simulink model "tc_dynamic_rl"  (R2026b)
settings: Solver=ode15s  StopTime=0.0015  MaxStep=1.9999999999999999e-07  RelTol=1e-06  AbsTol=1e-09
model workspace (MAT data in the model file):
  tcCommand = timeseries
  tcCommand.Name = 'unnamed'
  tcCommand.DataInfo = tsdata.datametadata
  tcCommand.DataInfo.Interpolation = tsdata.interpolation
  tcCommand.DataInfo.Interpolation.Fhandle : function handle (value not decoded)
  tcCommand.DataInfo.Interpolation.Name = 'linear'
  tcCommand.TimeInfo = tsdata.timemetadata
  tcCommand.TimeInfo.Length = 6
  tcCommand.TimeInfo.DuplicateTimes = 0
  tcCommand.TimeInfo.Time_ = [0; 5e-05; 0.0003; 0.0004; 0.0005; 0.0015]
  tcCommand.TimeInfo.Initialized = 1
  tcCommand.QualityInfo = tsdata.qualmetadata
  tcCommand.Data_ = [0; 1; 0; 1; 0; 0]
libraries: fl_lib x15, nesl_utility x10, ee_lib x3
settings Model: Creator=ganib  LastModifiedBy=ganib
settings SimscapeCC: SimscapeLogType=all  SimscapeNominalValues="[{\"value\":\"1\",\"unit\":\"A\"},{\"value\":\"1\",\"unit\":\"bar\"},{\"value\":\"1\",\"unit\":\"cm^2\"},{\"value\":\"1\",\"unit\":\"cm^3/s\"},{\"value\":\"1\",\"unit\":\"kJ/kg\"},{\"value\":\"1\",\"unit\":\"kW\"},{\"value\":\"1\",\"unit\":\"l\"},{\"value\":\"1\",\"unit\":\"N\"},{\"value\":\"1\",\"unit\":\"N*m\"},{\"value\":\"1\",\"unit\":\"V\"},{\"value\":\"0.001\",\"unit\":\"Wb\"}]"  SimscapeUseEnergyAccounting=off

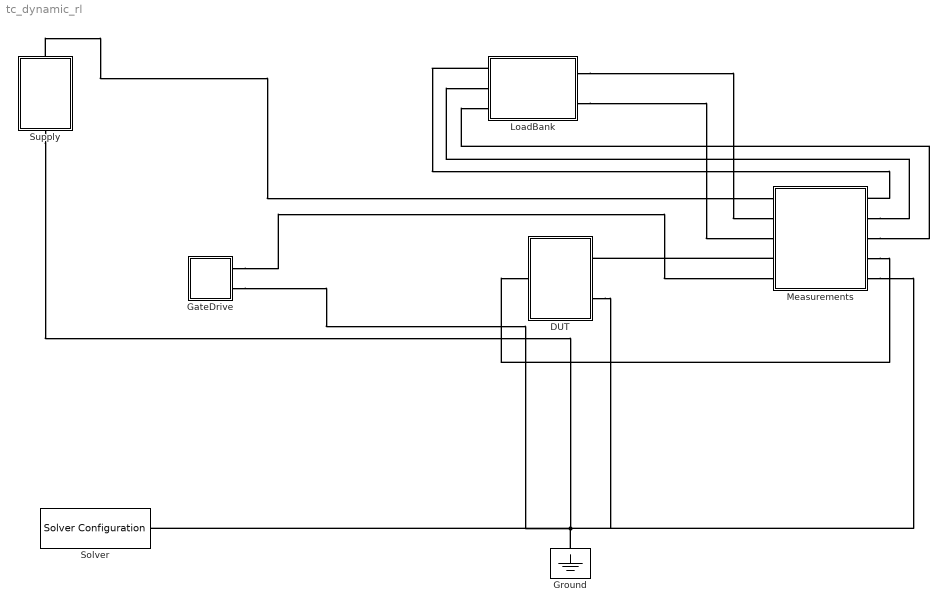
== system tc_dynamic_rl ==
  DUT : Subsystem
  GateDrive : Subsystem
  Ground : fl_lib/Electrical/Electrical Elements/Electrical Reference
  LoadBank : Subsystem
  Measurements : Subsystem
  Solver : nesl_utility/Solver Configuration  PhysicalDomain=network_engine_domain  SubClassName=solver  LeftPortType=input  RightPortType=generic  Tones=[]  Harmonics=[]  SimulateNoise=off  Profile=off  UseLocalSampling=off  EnableSwitchedLinearOptims=on  FrequencyDomain=off  UseCCode=off  RelTol=0.001  AbsTol=0.001  MinStep=1e-09  ToWorkspace=off  RevertToSquareIcSolve=off  NumHomotopyIterations=100  PhasorMode=off  PhasorModeNumHarmonics=1  ConsistencySolver=NEWTON_XTOL_AFTER_FTOL  CanonicalOrdering=CANONICAL  OptimizeIntermediates=OPTIMIZED  MulticoreSolverChoice=BACKWARD_EULER  IndexReductionMethod=DerivativeReplacement  DoDC=on  ResidualTolerance=1e-09  ConsistencyTolSource=GLOBAL  ConsistencyAbsTol=0.001  ConsistencyRelTol=0.001  ConsistencyTolFactor=0.001  UseLocalSolver=off  LocalSolverChoice=NE_BACKWARD_EULER_ADVANCER  ResolveIndetEquations=on  FunctionEvalNumThread=1  LocalSolverSampleTime=0.001  DoFixedCost=off  MaxNonlinIter=3  MaxModeIter=2  ComputeImpulses=off  ImpulseIterations=2  LinearAlgebra=auto  LinearAlgebraNumThread=0  EquationFormulation=NE_TIME_EF  DelaysMemoryBudget=1024  AutomaticFiltering=on  FilteringTimeConstant=0.001  PartitionStorageMethod=AS_NEEDED  PartitionMemoryBudget=1024  PartitionMethod=BALANCED  MultibodyUseLocalSolver=off  MultibodyLocalSolverChoice=ODE1  MultibodyLocalSolverSampleTime=0.001
  Supply : Subsystem
  connections:
  Ground/LConn1 -- Supply/RConn1 -- Measurements/RConn5 -- DUT/RConn2 -- GateDrive/RConn2 -- Solver/RConn1
  Supply/LConn1 -- Measurements/LConn1
  LoadBank/LConn1 -- Measurements/RConn1
  LoadBank/RConn1 -- Measurements/LConn2
  Measurements/RConn2 -- LoadBank/LConn2
  LoadBank/RConn2 -- Measurements/LConn3
  Measurements/RConn3 -- LoadBank/LConn3
  Measurements/LConn4 -- DUT/RConn1
  GateDrive/RConn1 -- Measurements/LConn5
  Measurements/RConn4 -- DUT/LConn1

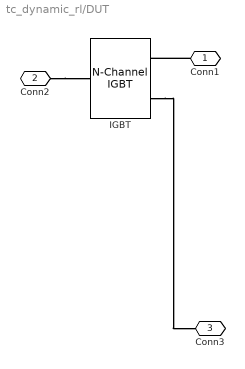
== system tc_dynamic_rl/DUT ==
  IGBT : ee_lib/Semiconductors & Converters/N-Channel IGBT  model_type=ee.enum.igbt.parameterization.equation  Ices=1.1501079949162614e-07 A  Vces=3300 V  Vth=6.3 V  Vce_sat=2.6 V  Ice_sat=1500 A  Vge_sat=15 V  Tmeas=25 degC  Vge_vec=[-1, 0, 2, 3, 5, 6, 7, 8, 10, 12, 15, 18, 20] V  Vce_vec=[0, .25, .5, .75, 1, 1.26, 1.51, 1.76, 2.01, 2.26, 2.51, 2.76, 3.01, 3.27, 3.52, 3.77, 4.02, 4.27, 4.52, 4.77] V  T_vec=[25, 125] degC  Ic_mat=[0, 0, 0, 0, 0, 0, 0, 0, 0, 0, 0, 0, 0, 0, 0, 0, 0, 0, 0, 0; 0, 0, 0, 0, 0, 0, 0, 0, 0, 0, 0, 0, 0, 0, 0, 0, 0, 0, 0, 0; 0, 0, 0, 0, 0, 0, 0, 0, 0, 0, 0, 0, 0, 0, 0, 0, 0, 0, 0, 0; 0, 0, 0, 0, 0, 0, 0, 0, 0, 0, 0, 0, 0, 0, 0, 0, 0, 0, 0, 0; 0, 0, 0, 0, 0, 0, 0, 0, 0, 0, 0, 0, 0, 0, 0, 0, 0, 0, 0, 0; 0, 0, 0, .81, 3.13, 4.97, 6.03, 6.53, 6.84, 7.01, 7.19, 7.32, 7.44, 7.55, 7.67, 7.78, 7.89, 8, 8.07, 8.07; 0, 0, 0, 1.07, 5.5, 12.93, 22.09, 29.14, 35.27, 38.97, 41.37, 43.08, 44.52, 45.45, 46.28, 46.85, 47.41, 47.76, 48.06, 48.36; 0, 0, 0, 1.1, 6.99, 16.51, 28.38, 41.53, 55.76, 69.08, 80.5, 89.56, 96.13, 101.45, 105.15, 107.99, 110.09, 111.87, 113.54, 114.95; 0, 0, 0, 1.36, 6.26, 17.43, 33.6, 50.43, 71.75, 93.61, 114.64, 134.42, 151.44, 164.25, 177.06, 189.88, 202.69, 215.51, 228.32, 241.14; 0, 0, 0, 1.42, 6.4, 18.7, 36.19, 55.23, 79.71, 106.22, 131.28, 156.62, 182.79, 208.97, 235.15, 261.32, 287.5, 313.67, 339.85, 366.02; 0, 0, 0, 1.45, 6.81, 20.01, 39.61, 60.63, 88.74, 117.7, 147.16, 191.87, 237.14, 282.42, 327.69, 372.96, 418.23, 463.5, 508.77, 554.04; 0, 0, 0, 1.49, 6.97, 20.55, 41.34, 64.15, 94.91, 126.1, 170.16, 233.77, 297.38, 360.98, 424.59, 488.19, 551.8, 615.4, 679.01, 742.62; 0, 0, 0, 1.5, 7.5, 20.96, 42.17, 66.19, 98.34, 131.14, 187.84, 263.46, 339.09, 414.72, 490.34, 565.97, 641.6, 717.22, 792.85, 868.48] A  Ic_mat_3D=zeros(13, 20, 2) A  C_param=ee.enum.igbt.capacitanceParam.fixedciss  C_GE=23.7 nF  C_GC=2.7 nF  C_CE=0 nF  C_ies=1.6400000000000001e-07 F  C_res=1.3999999999999999e-09 F  C_oes=1.0999999999999999e-08 F  C_GE_vec=[25, 31, 26.5, 24.9, 25, 24.9, 24.6, 24.7, 24.8] nF  C_GC_vec=[55, 9, 5.5, 3.1, 2.5, 2.1, 1.9, 1.8, 1.7] nF  C_Vge_vec=0 V  C_CE_vec=[5, 11, 6.5, 4.9, 3.5, 2.7, 2.1, 1.7, 1.4] nF  C_ies_vec=[80, 40, 32, 28, 27.5, 27, 26.5, 26.5, 26.5] nF  C_res_vec=[55, 9, 5.5, 3.1, 2.5, 2.1, 1.9, 1.8, 1.7] nF  C_oes_vec=[60, 20, 12, 8, 6, 4.8, 4, 3.5, 3.1] nF  C_Vce_vec=[0, 1, 2, 5, 10, 15, 20, 25, 30] V  charge_linearity_param=ee.enum.igbt.cgcLinearity.constant  C_OX=20 nF  V_C_OX=-5 V  TF=1.9999999999999999e-07 s  TT=0 us  LeadRc=0 Ohm  LeadRe=0 Ohm  LeadRg=0 Ohm  LC=0 nH  LE=0 nH  LG=0 nH  ec=1  VAF=200 V  RC=4.5e-05 Ohm  RE=4.5e-05 Ohm  RG=0.5 Ohm  BF=50  T_param=ee.enum.igbt.temperatureParameterization.IcesVce  Ices_T2=0.0040000000000000001 A  EG=1.11 eV  Vce_sat_T2=3.2 V  Tmeas2=125 degC  XTI=3  BEX=-1.5  RG_alpha=0 1/K  Tdevice=25 degC  Tdevice_3D=25 degC  ig_specify=off  ig_priority=None  ig=0 A  ig_nominal_specify=off  ig_nominal_value=1  ig_nominal_unit=A  ic_specify=off  ic_priority=None  ic=0 A  ic_nominal_specify=off  ic_nominal_value=1  ic_nominal_unit=A  vge_specify=off  vge_priority=None  vge=0 V  vge_nominal_specify=off  vge_nominal_value=1  vge_nominal_unit=V  vce_specify=off  vce_priority=None  vce=0 V  vce_nominal_specify=off  vce_nominal_value=1  vce_nominal_unit=V  v_Cge_specify=off  v_Cge_priority=High  v_Cge=0 V  v_Cge_nominal_specify=off  v_Cge_nominal_value=1  v_Cge_nominal_unit=V  v_Cce_specify=off  v_Cce_priority=High  v_Cce=0 V  v_Cce_nominal_specify=off  v_Cce_nominal_value=1  v_Cce_nominal_unit=V  thermal_network_parameterization=ee.enum.thermalNetworkTopology.junctionCase  Rth=[0, 10] K/W  Rth_Cauer=[1, 3, 10] K/W  Rth_Foster=[.08, .14, .22, .16] K/W  thermal_mass_parameterization=ee.enum.thermalNetwork.timeconstant  thermal_mass=[0, 1] J/K  thermal_mass_Cauer=[.1, .3, 1] J/K  thermal_mass_Foster=[.001, .005, .05, .5] J/K  thermal_time_constant=[0, 10] s  thermal_time_constant_Cauer=[1, 3, 10] s  thermal_time_constant_Foster=[7e-05, .0007, .01, .08] s  thermal_mass_initial_temperatures=[25, 25] degC  thermal_mass_initial_temperatures_Cauer=[25, 25, 25] degC  Tvec_initial_Foster=[25, 25, 25, 25] degC  Ic_vec1=[0, 10, 50, 100, 200, 400, 600] A  Vce_vec1=[0, 1.1, 1.3, 1.45, 1.75, 2.25, 2.7] V  Rmiller=0.1 Ohm  Goff=1e-5 1/Ohm  t_on=0.07 us  t_rise=0.7 us  t_off=0.2 us  t_fall=0.5 us  v_meas=300 V  vStartTurnOn_specify=off  vStartTurnOn_priority=None  vStartTurnOn=1 V  tStartTurnOn_specify=off  tStartTurnOn_priority=None  tStartTurnOn=0 s  vStartTurnOff_specify=off  vStartTurnOff_priority=None  vStartTurnOff=0.5 V  tStartTurnOff_specify=off  tStartTurnOff_priority=None  tStartTurnOff=0 s  Tj_vec1=[298.15, 398.15] K  Vce_mat1=[0, 1.1, 1.3, 1.45, 1.75, 2.25, 2.7; 0, 1, 1.15, 1.35, 1.7, 2.35, 3] V  Tj_vec_loss=[298.15, 398.15] K  Ic_vec_loss=[0, 10, 50, 100, 200, 400, 600] A  E_turn_on_mat1=[0, .2, 1, 2, 4, 8, 15; 0, .3, 1.3, 2.5, 5, 11, 18] * 1e-3 J  E_turn_off_mat1=[0, .3, 1.5, 3, 6, 15, 25; 0, .7, 3.3, 6.5, 13, 25, 35] * 1e-3 J  iStartTurnOff_specify=off  iStartTurnOff_priority=None  iStartTurnOff=0 A  Tdevice_specify=off  Tdevice_priority=None
  Conn1 : PMIOPort  Side=Right
  Conn2 : PMIOPort  Port=2  Side=Left
  Conn3 : PMIOPort  Port=3  Side=Right
  connections:
  Conn1/RConn1 -- IGBT/RConn1
  Conn2/RConn1 -- IGBT/LConn1
  IGBT/RConn2 -- Conn3/RConn1

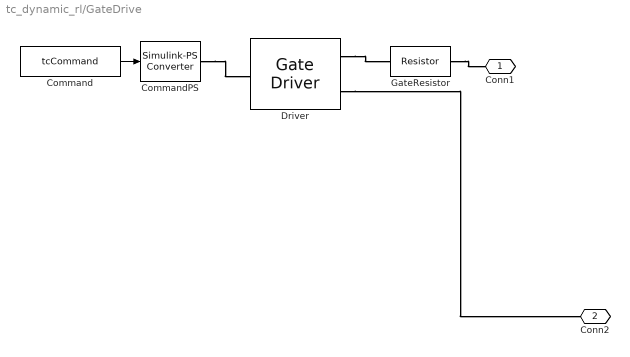
== system tc_dynamic_rl/GateDrive ==
  Command : FromWorkspace  VariableName=tcCommand  Interpolate=off  OutputAfterFinalValue=Holding final value
  CommandPS : nesl_utility/Simulink-PS Converter  PhysicalDomain=network_engine_domain  SubClassName=ps_input  LeftPortType=input  RightPortType=output  PseudoPeriodic=off  Frequencies=[]  NoiseDistribution=none  NoiseParameters=[]  Unit=1  AffineConversion=off  FilteringAndDerivatives=zero  SimscapeFilterOrder=1  InputFilterTimeConstant=0.001  UdotUserProvided=0
  Driver : ee_lib/Semiconductors & Converters/Gate Driver  port_option=ee.enum.controlport.ps  uHigh=2.0 V  uLow=0.8 V  uHighValue=0.7  uLowValue=0.3  vHigh=12 V  vLow=-15 V  tHigh=4.9999999999999998e-08 s  tLow=4.9999999999999998e-08 s  parameterization=ee.enum.semiconductors.gateDriverParam.outputImpedance  rHigh=2 Ohm  rLow=27 Ohm  tRise=20 ns  tFall=20 ns  cLoad=10 nF  ZonTime_specify=off  ZonTime_priority=None  ZonTime=0 s  ZoffTime_specify=off  ZoffTime_priority=None  ZoffTime=0 s
  GateResistor : fl_lib/Electrical/Electrical Elements/Resistor  R=0 Ohm  i_specify=off  i_priority=None  i=0 A  i_nominal_specify=off  i_nominal_value=1  i_nominal_unit=A  v_specify=off  v_priority=None  v=0 V  v_nominal_specify=off  v_nominal_value=1  v_nominal_unit=V
  Conn1 : PMIOPort  Side=Right
  Conn2 : PMIOPort  Port=2  Side=Right
  wires:
  Command/1 -> CommandPS/1
  connections:
  Driver/RConn1 -- GateResistor/LConn1
  CommandPS/RConn1 -- Driver/LConn1
  GateResistor/RConn1 -- Conn1/RConn1
  Driver/RConn2 -- Conn2/RConn1

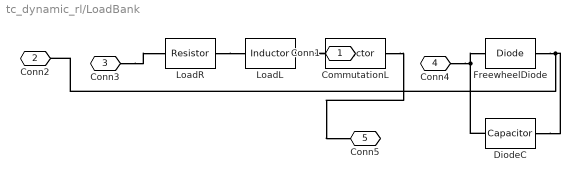
== system tc_dynamic_rl/LoadBank ==
  CommutationL : fl_lib/Electrical/Electrical Elements/Inductor  l=9.9999999999999995e-08 H  r=0.0001 Ohm  g=0 1/Ohm  i_specify=off  i_priority=None  i=0 A  i_nominal_specify=off  i_nominal_value=1  i_nominal_unit=A  v_specify=off  v_priority=None  v=0 V  v_nominal_specify=off  v_nominal_value=1  v_nominal_unit=V  i_L_specify=off  i_L_priority=High  i_L=0 A  i_L_nominal_specify=off  i_L_nominal_value=1  i_L_nominal_unit=A
  DiodeC : fl_lib/Electrical/Electrical Elements/Capacitor  c=1.0999999999999999e-08 F  r=1e-6 Ohm  g=0 1/Ohm  i_specify=off  i_priority=None  i=0 A  i_nominal_specify=off  i_nominal_value=1  i_nominal_unit=A  v_specify=off  v_priority=None  v=0 V  v_nominal_specify=off  v_nominal_value=1  v_nominal_unit=V  vc_specify=off  vc_priority=High  vc=0 V  vc_nominal_specify=off  vc_nominal_value=1  vc_nominal_unit=V
  FreewheelDiode : ee_lib/Semiconductors & Converters/Diode  Vf=0.5 V  Ron=0.0012 Ohm  Goff=1e-08 S  N_series=1  N_parallel=1  ZenerEnable=false  BV=30 V  Rz=0.3 Ohm  enable_fault_composite=simscape.enum.onoff.off  i_specify=off  i_priority=None  i=0 A  i_nominal_specify=off  i_nominal_value=1  i_nominal_unit=A  v_specify=off  v_priority=None  v=0 V  v_nominal_specify=off  v_nominal_value=1  v_nominal_unit=V  ModelType=ee.enum.diode.idealModelType.pwl  TableType=ee.enum.diode.tableType.IfMat  IfMat=[.07, .12, .19, 1.75, 4.24, 7.32, 11.2; .16, .3, .72, 2.14, 5.02, 8.35, 13.12] A  VfMat=[.9, 1.15, 1.25, 1.5, 1.75, 2.17, 2.6, 2.85; .58, .68, .75, 1.1, 1.38, 1.77, 2.27, 2.7] V  TjVec=[25, 125] degC  VfVec=[.5, .7, .9, 1.3, 1.7, 2.1, 2.5] V  IfVec=[.1, .2, .5, 1, 2, 4, 7, 10] A  IrMat=[1e-06, 2e-06, 5e-06, 1e-05, 2.5e-05, 5e-05, .0001; 2e-06, 5e-06, 1e-05, 4e-05, 8e-05, .0002, .0005] A  VrMat=[10, 100, 200, 250, 300, 325, 350; 10, 70, 160, 220, 270, 300, 320] V  VrVec=[10, 20, 40, 50, 70, 80, 100] V  IrVec=[1e-06, 2e-06, 5e-06, 1e-05, 2e-05, 5e-05, .0001] A  rec_loss_model=ee.enum.diode.reverseRecoveryModelTabulateUpTo3D.fixed  ErecVal=0 J  scaleWithIandV=true  ErecMat=zeros(2, 3) J  ErecMat3D=zeros(2, 3, 2) J  TjrecVec=[25, 125] degC  IfrecVec=[.1, 1, 10] A  IrecVal=10 A  VrecVal=10 V  VrecVec=[0, 100] V  tFilter=1 / 1000 / 100 s  thermal_network_parameterization=ee.enum.thermalNetworkTopology.junctionCase  Rth=[0, 10] K/W  Rth_Cauer=[1, 3, 10] K/W  Rth_Foster=[.08, .14, .22, .16] K/W  thermal_mass_parameterization=ee.enum.thermalNetwork.timeconstant  thermal_mass=[0, 1] J/K  thermal_mass_Cauer=[.1, .3, 1] J/K  thermal_mass_Foster=[.001, .005, .05, .5] J/K  thermal_time_constant=[0, 10] s  thermal_time_constant_Cauer=[1, 3, 10] s  thermal_time_constant_Foster=[7e-05, .0007, .01, .08] s  thermal_mass_initial_temperatures=[25, 25] degC  thermal_mass_initial_temperatures_Cauer=[25, 25, 25] degC  thermal_mass_initial_temperatures_Foster=[25, 25, 25, 25] degC  junction_thermal_mass=0.01 J/K  junction_temperature_specify=off  junction_temperature_priority=None  junction_temperature=25 degC  junction_temperature_nominal_specify=off  junction_temperature_nominal_value=1  junction_temperature_nominal_unit=degC  ThermalPort=false  ModelTypePhysical=ee.enum.diode.physicalModelType.exponential  prmExp=ee.enum.diode.expParam.useTwo  I12=[.0137, .545] A  V12=[.6, .7] V  IS=1e-12 A  ec=1  I1=0.0137 A  V1=0.6 V  RS=0 Ohm  C_param=ee.enum.diode.capParam.fixed  CJ=0 pF  CJ0=5 pF  Vvec=[.1, 10, 100] V  Cvec=[3.5, 1, .4] pF  VJ=1 V  Mgrad=0.5  FC=0.5  Q_param=ee.enum.diode.recoveryParam.off  iRM=-7.15 A  iF=4 A  didt=-750 A/us  trr_factor=3  trr=115 ns  Qrr=150 nA*s  Vr=-600 V  Ls=150 nH  Erec=0.03 J  TT=50 ns  tau=100 ns  T_param=ee.enum.diode.temperatureParam.off  Tmeas=25 degC  I1_T2=0.245 A  V1_T2=0.5 V  IS_T2=1.25e-7 A  Tmeas2=125 degC  EG_param=ee.enum.diode.egapParam.material_si  EG=1.11 eV  XTI_param=ee.enum.diode.xtiParam.pn  XTI=3  dBVdT=0 V/K  Tdevice=25 degC  i_capacitor_specify=off  i_capacitor_priority=None  i_capacitor=0 A  i_capacitor_nominal_specify=off  i_capacitor_nominal_value=1  i_capacitor_nominal_unit=A  Qj_specify=off  Qj_priority=None  Qj=0 C  Qj_nominal_specify=off  Qj_nominal_value=1  Qj_nominal_unit=uC
  LoadL : fl_lib/Electrical/Electrical Elements/Inductor  l=0.00029999999999999997 H  r=0 Ohm  g=0 1/Ohm  i_specify=off  i_priority=None  i=0 A  i_nominal_specify=off  i_nominal_value=1  i_nominal_unit=A  v_specify=off  v_priority=None  v=0 V  v_nominal_specify=off  v_nominal_value=1  v_nominal_unit=V  i_L_specify=off  i_L_priority=High  i_L=0 A  i_L_nominal_specify=off  i_L_nominal_value=1  i_L_nominal_unit=A
  LoadR : fl_lib/Electrical/Electrical Elements/Resistor  R=0.01 Ohm  i_specify=off  i_priority=None  i=0 A  i_nominal_specify=off  i_nominal_value=1  i_nominal_unit=A  v_specify=off  v_priority=None  v=0 V  v_nominal_specify=off  v_nominal_value=1  v_nominal_unit=V
  Conn1 : PMIOPort  Side=Right
  Conn2 : PMIOPort  Port=2  Side=Left
  Conn3 : PMIOPort  Port=3  Side=Left
  Conn4 : PMIOPort  Port=4  Side=Left
  Conn5 : PMIOPort  Port=5  Side=Right
  connections:
  DiodeC/LConn1 -- FreewheelDiode/LConn1 -- Conn4/RConn1
  LoadR/RConn1 -- LoadL/LConn1
  Conn3/RConn1 -- LoadR/LConn1
  FreewheelDiode/RConn1 -- Conn2/RConn1 -- DiodeC/RConn1
  Conn1/RConn1 -- CommutationL/LConn1 -- LoadL/RConn1
  CommutationL/RConn1 -- Conn5/RConn1

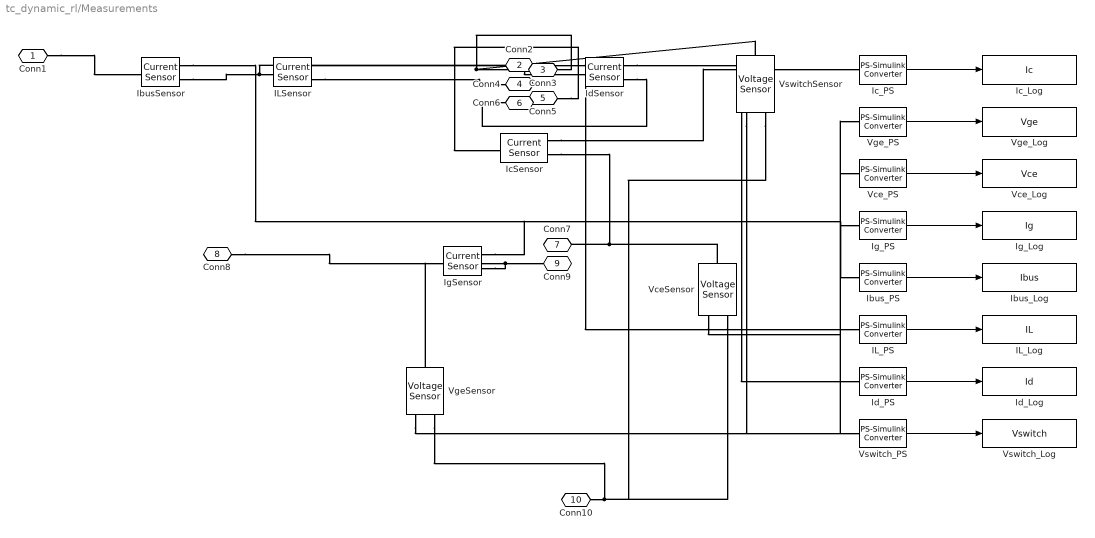
== system tc_dynamic_rl/Measurements ==
  ILSensor : fl_lib/Electrical/Electrical Sensors/Current Sensor
  IL_Log : ToWorkspace  VariableName=IL  SaveFormat=Timeseries  SampleTime=-1
  IL_PS : nesl_utility/PS-Simulink Converter  PhysicalDomain=network_engine_domain  SubClassName=ps_output  LeftPortType=input  RightPortType=output  PseudoPeriodic=off  Frequencies=[]  VectorFormat=inherit  Unit=A  AffineConversion=off
  IbusSensor : fl_lib/Electrical/Electrical Sensors/Current Sensor
  Ibus_Log : ToWorkspace  VariableName=Ibus  SaveFormat=Timeseries  SampleTime=-1
  Ibus_PS : nesl_utility/PS-Simulink Converter  PhysicalDomain=network_engine_domain  SubClassName=ps_output  LeftPortType=input  RightPortType=output  PseudoPeriodic=off  Frequencies=[]  VectorFormat=inherit  Unit=A  AffineConversion=off
  IcSensor : fl_lib/Electrical/Electrical Sensors/Current Sensor
  Ic_Log : ToWorkspace  VariableName=Ic  SaveFormat=Timeseries  SampleTime=-1
  Ic_PS : nesl_utility/PS-Simulink Converter  PhysicalDomain=network_engine_domain  SubClassName=ps_output  LeftPortType=input  RightPortType=output  PseudoPeriodic=off  Frequencies=[]  VectorFormat=inherit  Unit=A  AffineConversion=off
  IdSensor : fl_lib/Electrical/Electrical Sensors/Current Sensor
  Id_Log : ToWorkspace  VariableName=Id  SaveFormat=Timeseries  SampleTime=-1
  Id_PS : nesl_utility/PS-Simulink Converter  PhysicalDomain=network_engine_domain  SubClassName=ps_output  LeftPortType=input  RightPortType=output  PseudoPeriodic=off  Frequencies=[]  VectorFormat=inherit  Unit=A  AffineConversion=off
  IgSensor : fl_lib/Electrical/Electrical Sensors/Current Sensor
  Ig_Log : ToWorkspace  VariableName=Ig  SaveFormat=Timeseries  SampleTime=-1
  Ig_PS : nesl_utility/PS-Simulink Converter  PhysicalDomain=network_engine_domain  SubClassName=ps_output  LeftPortType=input  RightPortType=output  PseudoPeriodic=off  Frequencies=[]  VectorFormat=inherit  Unit=A  AffineConversion=off
  VceSensor : fl_lib/Electrical/Electrical Sensors/Voltage Sensor
  Vce_Log : ToWorkspace  VariableName=Vce  SaveFormat=Timeseries  SampleTime=-1
  Vce_PS : nesl_utility/PS-Simulink Converter  PhysicalDomain=network_engine_domain  SubClassName=ps_output  LeftPortType=input  RightPortType=output  PseudoPeriodic=off  Frequencies=[]  VectorFormat=inherit  Unit=V  AffineConversion=off
  VgeSensor : fl_lib/Electrical/Electrical Sensors/Voltage Sensor
  Vge_Log : ToWorkspace  VariableName=Vge  SaveFormat=Timeseries  SampleTime=-1
  Vge_PS : nesl_utility/PS-Simulink Converter  PhysicalDomain=network_engine_domain  SubClassName=ps_output  LeftPortType=input  RightPortType=output  PseudoPeriodic=off  Frequencies=[]  VectorFormat=inherit  Unit=V  AffineConversion=off
  VswitchSensor : fl_lib/Electrical/Electrical Sensors/Voltage Sensor
  Vswitch_Log : ToWorkspace  VariableName=Vswitch  SaveFormat=Timeseries  SampleTime=-1
  Vswitch_PS : nesl_utility/PS-Simulink Converter  PhysicalDomain=network_engine_domain  SubClassName=ps_output  LeftPortType=input  RightPortType=output  PseudoPeriodic=off  Frequencies=[]  VectorFormat=inherit  Unit=V  AffineConversion=off
  Conn1 : PMIOPort  Side=Left
  Conn2 : PMIOPort  Port=2  Side=Right
  Conn3 : PMIOPort  Port=3  Side=Left
  Conn4 : PMIOPort  Port=4  Side=Right
  Conn5 : PMIOPort  Port=5  Side=Left
  Conn6 : PMIOPort  Port=6  Side=Right
  Conn7 : PMIOPort  Port=7  Side=Left
  Conn8 : PMIOPort  Port=8  Side=Left
  Conn9 : PMIOPort  Port=9  Side=Right
  Conn10 : PMIOPort  Port=10  Side=Right
  wires:
  Ic_PS/1 -> Ic_Log/1
  Vswitch_PS/1 -> Vswitch_Log/1
  Id_PS/1 -> Id_Log/1
  Vge_PS/1 -> Vge_Log/1
  Vce_PS/1 -> Vce_Log/1
  Ibus_PS/1 -> Ibus_Log/1
  Ig_PS/1 -> Ig_Log/1
  IL_PS/1 -> IL_Log/1
  connections:
  IbusSensor/RConn2 -- Conn2/RConn1 -- ILSensor/LConn1
  VswitchSensor/RConn1 -- Vswitch_PS/LConn1
  IdSensor/RConn2 -- Conn6/RConn1
  ILSensor/RConn1 -- IL_PS/LConn1
  IbusSensor/RConn1 -- Ibus_PS/LConn1
  IdSensor/RConn1 -- Id_PS/LConn1
  VswitchSensor/LConn1 -- Conn3/RConn1 -- IdSensor/LConn1
  Conn8/RConn1 -- IgSensor/LConn1
  VgeSensor/LConn1 -- Conn9/RConn1 -- IgSensor/RConn2
  IcSensor/RConn1 -- Ic_PS/LConn1
  IcSensor/RConn2 -- Conn7/RConn1 -- VceSensor/LConn1
  ILSensor/RConn2 -- Conn4/RConn1
  IgSensor/RConn1 -- Ig_PS/LConn1
  VceSensor/RConn1 -- Vce_PS/LConn1
  VgeSensor/RConn1 -- Vge_PS/LConn1
  Conn1/RConn1 -- IbusSensor/LConn1
  Conn5/RConn1 -- IcSensor/LConn1
  Conn10/RConn1 -- VceSensor/RConn2 -- VswitchSensor/RConn2 -- VgeSensor/RConn2

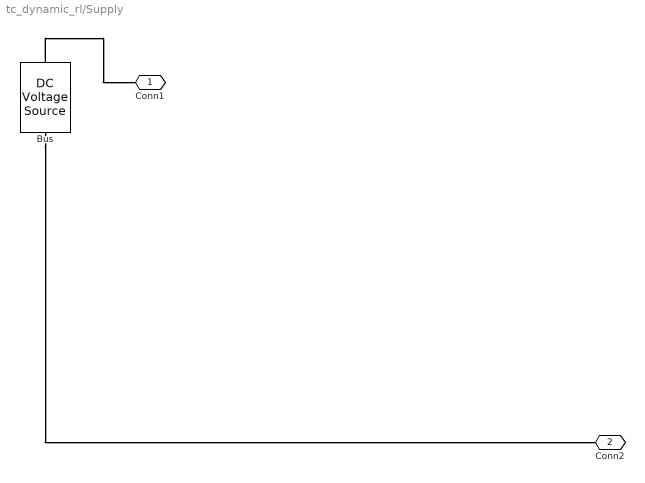
== system tc_dynamic_rl/Supply ==
  Bus : fl_lib/Electrical/Electrical Sources/DC Voltage Source  v0=1800 V
  Conn1 : PMIOPort  Side=Left
  Conn2 : PMIOPort  Port=2  Side=Right
  connections:
  Bus/LConn1 -- Conn1/RConn1
  Bus/RConn1 -- Conn2/RConn1
